simulink model "simulink_model"  (R2026b)
settings: Solver=VariableStepAuto
libraries: simulink x1
settings Model: Creator=Gabe  LastModifiedBy=Gabe

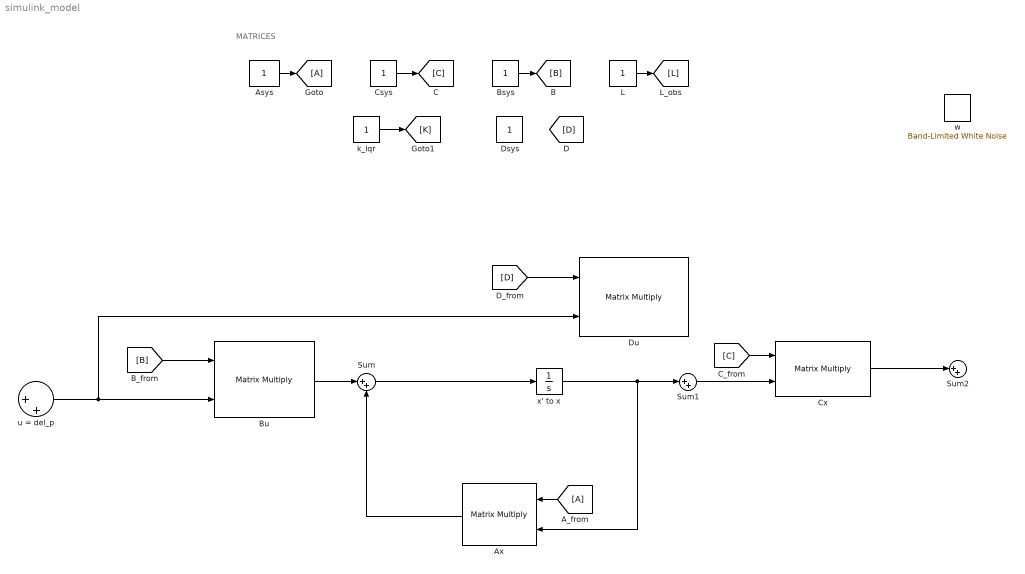
== system simulink_model ==
  note: MATRICES
  A_from : From
  Asys : Constant
  Ax : Product  Multiplication=Matrix(*)
  Bsys : Constant
  Bu : Product  Multiplication=Matrix(*)
  Csys : Constant
  Cx : Product  Multiplication=Matrix(*)
  Dsys : Constant
  Du : Product  Multiplication=Matrix(*)
  Goto : Goto
  L : Constant
  Sum : Sum  Inputs=|++
  Sum1 : Sum  Inputs=|++
  Sum2 : Sum  Inputs=|++
  k_lqr : Constant
  u = del_p : Sum  Inputs=|++
  w : simulink/Sources/Band-Limited White Noise  Cov=[0.1]  Ts=0.1  seed=[23341]
  x' to x : Integrator
  wires:
  Asys/1 -> Goto/1
  Csys/1 -> [C]
  Bsys/1 -> [B]
  L/1 -> [L]
  k_lqr/1 -> [K]
  A_from/1 -> Ax/1
  Sum/1 -> x' to x/1
  x' to x/1 -> Ax/2, Sum1/1
  Sum1/1 -> Cx/2
  [C] -> Cx/1
  Cx/1 -> Sum2/1
  [B] -> Bu/1
  Ax/1 -> Sum/2
  [D] -> Du/1
  Bu/1 -> Sum/1
  u = del_p/1 -> Du/2, Bu/2
